simulink model "Horizontal1804"  (R2026b)
settings: Solver=FixedStepDiscrete  StopTime=inf  FixedStep=Official.Step
PostLoadFcn:
  | run(fullfile(fileparts(get_param('StampFly_IMU400','FileName')),'config','startup.m'));
InitFcn:
  | init_imu_flight;
undefined symbols (not defined in the file): Official
libraries: slpidlib x7, simulink x4, mspfiltlib x1
(part 1 of 5)
settings Model: SILPILModeSetting=veronly  Creator=tyasukaw  LastModifiedBy=tyasukaw
settings SolverCC: AutoInsertRateTranBlk=on
settings OptimizationCC: DifferentSizesBufferReuse=on  EfficientTunableParamExpr=on  EnhancedBackFolding=on  MaxStackSize=64  OptimizationCustomize=off  OptimizeBlockOrder=speed  PassReuseOutputArgsAs=Individual arguments  RemoveInternalMemoryZeroInit=on  RemoveRootLevelIOMemoryZeroInit=on
settings DebuggingCC: ParameterTunabilityLossMsg=error
settings HardwareCC: ProdHWDeviceType=ARM Compatible->ARM Cortex  ProdLargestAtomicFloat=Double  ProdLargestAtomicInteger=Long
settings SFSimCC: MATLABDynamicMemAlloc=off
settings RTWCC: BuildConfiguration=Faster Runs  DataTypeReplacement=CDataTypesFixedWidth  Description=Embedded Coder  HardwareBoard=ESP32-S3 Series (Arduino Compatible)  SystemTargetFile=ert.tlc  TLCOptions="-aInlineSetEventsForThisBaseRateFcn=TLC_FALSE -aSuppressMultiTaskScheduler=TLC_FALSE  -aRateBasedStepFcn=0"  TemplateMakefile=ert_default_tmf  Toolchain=ESP32
settings CodeAppCC: ForceParamTrailComments=on  IgnoreCustomStorageClasses=off  InsertBlockDesc=on  OperatorAnnotations=on  SFDataObjDesc=on  SimulinkDataObjDesc=on
settings ERTTargetCC: CombineSignalStateStructs=on  ExtModeAutomaticAllocSize=off  ExtModeIntrfLevel=Level2 - Open  ExtModeMexFile=ext_xcp  ExtModeStaticAlloc=on  MaxIdInt16=INT16_MAX  MaxIdInt32=INT32_MAX  MaxIdInt64=INT64_MAX  MaxIdInt8=INT8_MAX  MaxIdUint16=UINT16_MAX  MaxIdUint32=UINT32_MAX  MaxIdUint64=UINT64_MAX  MaxIdUint8=UINT8_MAX  MinIdInt16=INT16_MIN  MinIdInt32=INT32_MIN  MinIdInt64=INT64_MIN  MinIdInt8=INT8_MIN  SupportContinuousTime=on  SupportVariableSizeSignals=on

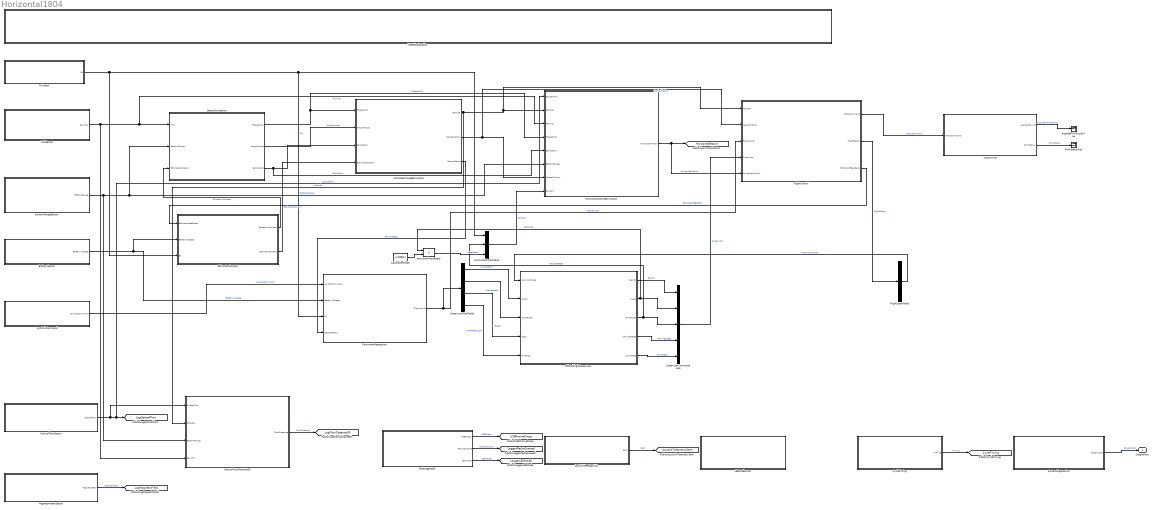
== system Horizontal1804 ==
  AppliedPWMCountsTap : Terminator
      settings: Description=AppliedPWMCountsTap：使用しない観測出力をここで終端します。接続された制御信号を変更しません。
  AttitudeAltitudeEstimation : Subsystem  Description=IMU Filter で姿勢・補正済み角速度、MATLAB Function の AltitudeKalman で高度・鉛直速度を推定します。状態フラグと推定診断をまとめ、ログ用 Goto をこの階層から公開します。
      mask help: IMU Filter で姿勢・補正済み角速度、MATLAB Function の AltitudeKalman で高度・鉛直速度を推定します。状態フラグと推定診断をまとめ、ログ用 Goto をこの階層から公開します。
      mask Display: disp('AttitudeAltitudeEstimation');port_label('input',1,'FilteredIMU');port_label('input',2,'HeightInputs');port_label('input',3,'Calibration');port_label('input',4,'EstimatorContext');port_label('output',1,'Attitude');port_label('output',2,'VerticalMotion');port_label('output',3,'SensorStatus');
  BatterySensor : Subsystem  Description=電池電圧 [V] と読み出し有効性を取得します。I2C 使用中は前回値を保持し、ReadValid=0 を公開します。
      mask help: 電池電圧 [V] と読み出し有効性を取得します。I2C 使用中は前回値を保持し、ReadValid=0 を公開します。
      mask Display: disp('BatterySensor');port_label('output',1,'BatteryVoltage');
  BottomRangeSensor : Subsystem  Description=下向き ToF の初期化完了後は Mode に依存せず取得します。距離 [mm] と Fresh を BottomRange バスへまとめ、Status と診断は Goto で公開します。Fresh は 400 Hz の読み出しではなく新しい測定結果の到着を示します。前方センサーは未使用です。
      mask help: 下向き ToF の初期化完了後は Mode に依存せず取得します。距離 [mm] と Fresh を BottomRange バスへまとめ、Status と診断は Goto で公開します。Fresh は 400 Hz の読み出しではなく新しい測定結果の到着を示します。前方センサーは未使用です。
      mask Display: disp('BottomRangeSensor');port_label('output',1,'BottomRange');
  CalibrationMode : Constant  Description=CalibrationMode：水平推定・制御のデータと実行条件を選択・結合します。2軸の順序は局所X（基準機首）、Y（右）です。  Value=uint8(1)
  CommandPreparation : Subsystem  Description=操縦指令、電池電圧、実測 dt、センサーフラグを名前付きバスへまとめます。Stateflow と飛行制御へ同じ入力を渡し、ログ用の観測も公開します。
      mask help: 操縦指令、電池電圧、実測 dt、センサーフラグを名前付きバスへまとめます。Stateflow と飛行制御へ同じ入力を渡し、ログ用の観測も公開します。
      mask Display: disp('CommandPreparation');port_label('input',1,'JoystickCommand');port_label('input',2,'BatteryVoltage');port_label('input',3,'Dt');port_label('input',4,'SensorStatus');port_label('output',1,'FlightInputs');
  CycleTiming : Subsystem  Description=ログとモーター適用後の処理時間・周期間隔を観測します。制御値を変更せず、計測位置を信号依存で固定します。
      mask help: ログとモーター適用後の処理時間・周期間隔を観測します。制御値を変更せず、計測位置を信号依存で固定します。
      mask Display: disp('CycleTiming');port_label('output',1,'Timing');
  DataLogging50 : Subsystem  Description=全ログ入力を50 Hzで同時に保存し、400 Hzタスク内で指令補足を2.5 ms後、センサー補足を5 ms後、通常ログを10 ms後に作成・送信します。水平補足は7.5 ms後です。保存時刻・Sequence・項目順・型・CRCで対応づけます。Channelは操縦受信・ログ受信機と同じ専用CHです。
      mask help: 生センサー・推定・制御・追加センサーを名前付き From で取得し、50 Hz の SFI8/SFIX/SFIY ログを生成して送信します。型・順序・CRC は維持します。Channel は RadioUSBTransport50 の設定画面で操縦側と揃えます。
      mask Display: disp('DataLogging50');port_label('output',1,'USBDrops');port_label('output',2,'RadioQueued');port_label('output',3,'LEDMode');
  EstimatorContext : Subsystem  Description=前周期のモード、高度制御許可、姿勢・待機リセットを 1 周期保持して推定器へ渡します。状態更新順序と代数ループ回避に必要な遅延です。
      mask help: 前周期のモード、高度制御許可、姿勢・待機リセットを 1 周期保持して推定器へ渡します。状態更新順序と代数ループ回避に必要な遅延です。
      mask Display: disp('EstimatorContext');port_label('input',1,'EstimatorFeedback');port_label('input',2,'BatteryVoltage');port_label('input',3,'Dt');port_label('output',1,'CorrectionContext');port_label('output',2,'EstimatorContext');
  FlightControl : Subsystem  Description=最上位 Stateflow の指令と姿勢・高度を受け、離着陸、7 個の PID、モーター配分を計算します。出力は Duty・PWM Counts、飛行状態、次周期の推定器コンテキストです。状態ログもこの階層に含みます。
      mask help: 最上位 Stateflow の指令と姿勢・高度を受け、離着陸、7 個の PID、モーター配分を計算します。出力は Duty・PWM Counts、飛行状態、次周期の推定器コンテキストです。状態ログもこの階層に含みます。
      mask Display: disp('FlightControl');port_label('input',1,'Attitude');port_label('input',2,'VerticalMotion');port_label('input',3,'FlightInputs');port_label('input',4,'Supervisor');port_label('input',5,'HorizontalMotion');port_label('output',1,'MotorCommand');port_label('output',2,'FlightStatus');port_label('output',3,'EstimatorFeedback');
  FlightStateFields : BusSelector  Description=FlightStateFields：バスから PreviousMode を選びます。元のベクトルの成分順序は変更しません。  OutputSignals=PreviousMode
  HorizontalContextBus : BusCreator  Description=HorizontalContextBus：水平推定・制御のデータと実行条件を選択・結合します。2軸の順序は局所X（基準機首）、Y（右）です。  Inputs=3  OutDataTypeStr=Bus: HorizontalContextBus  NonVirtualBus=on
      settings: InheritFromInputs=off
  HorizontalMotionEstimation : Subsystem  Description=HorizontalMotionEstimation：水平推定・制御のデータと実行条件を選択・結合します。2軸の順序は局所X（基準機首）、Y（右）です。
      mask help: 水平推定：フロー時刻に同期した角速度積分、ToFと姿勢による投影、品質と鮮度の確認を行います。局所Xは基準機首、Yは右です。
      mask Display: disp('HorizontalMotionEstimation');port_label('input',1,'OpticalFlow');port_label('input',2,'Attitude');port_label('input',3,'RawIMU');port_label('input',4,'FilteredIMU');port_label('input',5,'Calibration');port_label('input',6,'BottomRange');port_label('input',7,'VerticalMotion');port_label('input',8,'Context');port_label('output',1,'HorizontalMotion');
  HorizontalPoseReady : RelationalOperator  Description=HorizontalPoseReady：水平推定・制御のデータと実行条件を選択・結合します。2軸の順序は局所X（基準機首）、Y（右）です。  Operator=>  OutDataTypeStr=boolean  RndMeth=Simplest  InputSameDT=off
  IMUSensor : Subsystem  Description=BMI270 の生加速度・角速度を XYZ のままバスへまとめます。センサー座標であり、単位は m/s²・rad/s。温度と Fresh は名前付き Goto でログへ公開します。
      mask help: BMI270 の生加速度・角速度を XYZ のままバスへまとめます。センサー座標であり、単位は m/s²・rad/s。温度と Fresh は名前付き Goto でログへ公開します。
      mask Display: disp('IMUSensor');port_label('output',1,'RawIMU');
  JoystickCommand : Subsystem  Description=公式 JoyStick から通常飛行の指令を受信し、操縦バスと診断を公開します。Flip 用押し込みボタンは使用しません。専用 Channel は内部の BasicJoystick で設定します。
      mask help: 公式 JoyStick から通常飛行の指令を受信し、操縦バスと診断を公開します。Flip 用押し込みボタンは使用しません。専用 Channel は内部の BasicJoystick で設定します。
      mask Display: disp('JoystickCommand');port_label('output',1,'JoystickCommand');
  JoystickFeedback40 : Subsystem  Description=公式 JoyStick の画面へ姿勢・高度・電池・制御状態を 40 Hz で返信します。通常ログとは別の公式 120 byte 形式です。
      mask help: 公式 JoyStick の画面へ姿勢・高度・電池・制御状態を 40 Hz で返信します。通常ログとは別の公式 120 byte 形式です。
      mask Display: disp('JoystickFeedback40');port_label('output',1,'Sent');
  LEDAndBuzzer : Subsystem  Description=飛行状態・電池・通信・姿勢リセット要求から LED と音を決め、出力キューへ渡します。機体ボタンの押下・解放による再起動もここで扱います。
      mask help: 飛行状態・電池・通信・姿勢リセット要求から LED と音を決め、出力キューへ渡します。機体ボタンの押下・解放による再起動もここで扱います。
      mask Display: disp('LEDAndBuzzer');
  MagnetometerSensor : Subsystem  Description=BMM150 の磁場 XYZ [μT] と有効性・Fresh・診断を取得します。センサー座標を保ってログへ渡し、姿勢推定・制御には使いません。
      mask help: BMM150 の磁場 XYZ [μT] と有効性・Fresh・診断を取得します。センサー座標を保ってログへ渡し、姿勢推定・制御には使いません。
      mask Display: disp('MagnetometerSensor');port_label('output',1,'MagneticField');
  ModelExplanation : Subsystem  Description=StampFly の学習用実装。400 Hz でセンサー取得→校正→姿勢・高度推定→離着陸と 7 PID→4 モーターへ処理します。Flip はありません。最上位 Stateflow がモードを管理し、下段は観測・記録・状態表示です。
      mask help: StampFly の学習用実装。400 Hz でセンサー取得→校正→姿勢・高度推定→離着陸と 7 PID→4 モーターへ処理します。Flip はありません。最上位 Stateflow がモードを管理し、下段は観測・記録・状態表示です。
      mask Display: disp(sprintf('StampFly IMU Filter / 400 Hz\nセンサー取得 → 校正・前処理 → 姿勢・高度推定 → PID → モーター\n飛行モードは最上位のStateflowで管理。下段は観測・記録・状態表示。'));
  MotorWrite : Subsystem  Description=8 bit の Counts を実機モーターへ適用します。順序 [FR, FL, RR, RL]、GPIO [42, 5, 41, 10]、150 kHz 指定です。実適用 Counts と PWM 診断を Goto で公開します。
      mask help: 8 bit の Counts を実機モーターへ適用します。順序 [FR, FL, RR, RL]、GPIO [42, 5, 41, 10]、150 kHz 指定です。実適用 Counts と PWM 診断を Goto で公開します。
      mask Display: disp('MotorWrite');port_label('input',1,'MotorCommand');port_label('output',1,'AppliedCounts');port_label('output',2,'PWMStatus');
  OfficialFlightSupervisor : Stateflow chart  Description=最上位の飛行状態管理です。前周期 Mode、操縦ボタン、新パケット、異常フラグ、姿勢リセットを受け、校正・待機・飛行・着陸の分岐と推定器リセットを決めます。  TreatAsAtomicUnit=on
      mask help: 最上位の飛行状態管理です。前周期 Mode、操縦ボタン、新パケット、異常フラグ、姿勢リセットを受け、校正・待機・飛行・着陸の分岐と推定器リセットを決めます。
  OpticalFlowDistance50 : Subsystem  Description=生の累積光学フロー、姿勢、角速度、下向き ToF から平面上の東・北移動距離を 50 Hz で作ります。回転補償と品質判定を行い、無効な区間は位置を保持します。385 count/rad は初期値です。
      mask help: 生の累積光学フロー、姿勢、角速度、下向き ToF から平面上の東・北移動距離を 50 Hz で作ります。回転補償と品質判定を行い、無効な区間は位置を保持します。385 count/rad は初期値です。
      mask Display: disp('OpticalFlowDistance50');port_label('input',1,'OpticalFlow');port_label('input',2,'Attitude');port_label('input',3,'BottomRange');port_label('input',4,'RawIMU');port_label('output',1,'FlowDistance');
  OpticalFlowSensor : Subsystem  Description=PMW3901 の生 2 軸差分・品質・診断・累積カウントを取得します。表示・記録専用で、水平位置制御へは戻しません。
      mask help: PMW3901 の生 2 軸差分・品質・診断・累積カウントを取得します。表示・記録専用で、水平位置制御へは戻しません。
      mask Display: disp('OpticalFlowSensor');port_label('output',1,'OpticalFlow');
  PWMStatusTap : Terminator
      settings: Description=PWMStatusTap：使用しない観測出力をここで終端します。接続された制御信号を変更しません。
  SensorCorrection : Subsystem  Description=センサー座標から機体 XYZ へ変換し、800 周期の静止校正とフィルターを行います。加速度 XYZ・角速度 XYZ の順を維持し、ToF の保持・外れ値処理と鉛直加速度もまとめます。推定用の前処理は Mode 0, 1 で保持します。
      mask help: センサー座標から機体 XYZ へ変換し、800 周期の静止校正とフィルターを行います。加速度 XYZ・角速度 XYZ の順を維持し、ToF の保持・外れ値処理と鉛直加速度もまとめます。推定用の前処理は Mode 0, 1 で保持します。
      mask Display: disp('SensorCorrection');port_label('input',1,'IMU');port_label('input',2,'BottomRange');port_label('input',3,'EstimatorContext');port_label('output',1,'FilteredIMU');port_label('output',2,'HeightInputs');port_label('output',3,'Calibration');
  SupervisorCommandBus : BusCreator  Description=SupervisorCommandBus：異なる単位・型を持つ関連信号を名前付きバスにまとめます。入力線の信号名が項目名です。  Inputs=5
  SupervisorPilotFields : BusSelector  Description=SupervisorPilotFields：バスから ArmButton,NewPacket,Flags,AHRSRequest を選びます。元のベクトルの成分順序は変更しません。  OutputSignals=ArmButton,NewPacket,Flags,AHRSRequest
  SystemDiagnostics : Subsystem  Description=各機能の診断 From を型付き名前付きバスへまとめます。50 Hz/40 Hz の値を必要な箇所で保持し、全体の診断出力へ渡します。
      mask help: 各機能の診断 From を型付き名前付きバスへまとめます。50 Hz/40 Hz の値を必要な箇所で保持し、全体の診断出力へ渡します。
      mask Display: disp('SystemDiagnostics');port_label('output',1,'Diagnostics');
  TickStart : Subsystem  Description=400 Hz 周期の開始時刻、実測 dt、タイマー診断を取得し、秒への時刻変換と Goto 公開をこの階層でまとめます。
      mask help: 400 Hz 周期の開始時刻、実測 dt、タイマー診断を取得し、秒への時刻変換と Goto 公開をこの階層でまとめます。
      mask Display: disp('TickStart');port_label('output',1,'Dt');
  Diagnostics : Outport  OutDataTypeStr=Bus: OfficialDiagnosticBus  BusOutputAsStruct=on
  tag scope: CycleTiming=global, HorizontalMotion=global, JoystickTelemetrySent=global, LogFlowDistance50=global, LogMagneticField=global, LogOpticalFlow=global, LoggerLEDMode=global, LoggerRadioQueued=global, USBFrameDrops=global
  wires:
  JoystickFeedback40/1(Sent) -> [JoystickTelemetrySent]  "Sent"
  CycleTiming/1(Timing) -> [CycleTiming]  "Timing"
  SystemDiagnostics/1(Diagnostics) -> Diagnostics/1  "Diagnostics"
  DataLogging50/1(USBDrops) -> [USBFrameDrops]  "USBDrops"
  DataLogging50/2(RadioQueued) -> [LoggerRadioQueued]  "RadioQueued"
  DataLogging50/3(LEDMode) -> [LoggerLEDMode]  "LEDMode"
  SupervisorCommandBus/1 -> FlightControl/4(Supervisor)  "Supervisor"
  OfficialFlightSupervisor/5(connected) -> SupervisorCommandBus/5  "Connected"
  OfficialFlightSupervisor/4(parkingReset) -> SupervisorCommandBus/4  "ParkingReset"
  OfficialFlightSupervisor/1(branch) -> SupervisorCommandBus/1  "Branch"
  SupervisorPilotFields/4 -> OfficialFlightSupervisor/5(ahrsFlag)  "<AHRSRequest>"
  SupervisorPilotFields/3 -> OfficialFlightSupervisor/4(flags)  "<Flags>"
  SupervisorPilotFields/2 -> OfficialFlightSupervisor/3(newPacket)  "<NewPacket>"
  SupervisorPilotFields/1 -> OfficialFlightSupervisor/2(button)  "<ArmButton>"
  FlightStateFields/1 -> OfficialFlightSupervisor/1(previousMode)  "<PreviousMode>"
  FlightControl/2(FlightStatus) -> FlightStateFields/1  "FlightStatus"
  FlightControl/1(MotorCommand) -> MotorWrite/1(MotorCommand)  "MotorCommand"
  MotorWrite/1(AppliedCounts) -> AppliedPWMCountsTap/1  "AppliedPWMCounts"
  MotorWrite/2(PWMStatus) -> PWMStatusTap/1  "PWMStatus"
  AttitudeAltitudeEstimation/3(SensorStatus) -> CommandPreparation/4(SensorStatus)  "SensorStatus"
  CommandPreparation/1(FlightInputs) -> SupervisorPilotFields/1, FlightControl/3(FlightInputs)  "FlightInputs"
  JoystickCommand/1(JoystickCommand) -> CommandPreparation/1(JoystickCommand)  "JoystickCommand"
  FlightControl/3(EstimatorFeedback) -> EstimatorContext/1(EstimatorFeedback)  "EstimatorFeedback"
  EstimatorContext/2(EstimatorContext) -> AttitudeAltitudeEstimation/4(EstimatorContext)  "EstimatorContext"
  OpticalFlowDistance50/1(FlowDistance) -> [LogFlowDistance50]  "FlowDistance"
  MagnetometerSensor/1(MagneticField) -> [LogMagneticField]  "MagneticField"
  CalibrationMode/1 -> HorizontalPoseReady/2
  EstimatorContext/1(CorrectionContext) -> SensorCorrection/3(EstimatorContext)  "CorrectionContext"
  BatterySensor/1(BatteryVoltage) -> CommandPreparation/2(BatteryVoltage), EstimatorContext/2(BatteryVoltage)  "BatteryVoltage"
  OfficialFlightSupervisor/2(mode) -> SupervisorCommandBus/2, HorizontalPoseReady/1  "PreMode"
  SensorCorrection/2(HeightInputs) -> AttitudeAltitudeEstimation/2(HeightInputs)  "HeightInputs"
  HorizontalMotionEstimation/1(HorizontalMotion) -> [HorizontalMotion], FlightControl/5(HorizontalMotion)  "HorizontalMotion"
  AttitudeAltitudeEstimation/2(VerticalMotion) -> FlightControl/2(VerticalMotion), HorizontalMotionEstimation/7(VerticalMotion)  "VerticalMotion"
  SensorCorrection/1(FilteredIMU) -> AttitudeAltitudeEstimation/1(FilteredIMU), HorizontalMotionEstimation/4(FilteredIMU)  "FilteredIMU"
  SensorCorrection/3(Calibration) -> AttitudeAltitudeEstimation/3(Calibration), HorizontalMotionEstimation/5(Calibration)  "Calibration"
  BottomRangeSensor/1(BottomRange) -> HorizontalMotionEstimation/6(BottomRange), SensorCorrection/2(BottomRange), OpticalFlowDistance50/3(BottomRange)  "BottomRange"
  OpticalFlowSensor/1(OpticalFlow) -> HorizontalMotionEstimation/1(OpticalFlow), [LogOpticalFlow], OpticalFlowDistance50/1(OpticalFlow)  "OpticalFlow"
  IMUSensor/1(RawIMU) -> SensorCorrection/1(IMU), HorizontalMotionEstimation/3(RawIMU), OpticalFlowDistance50/4(RawIMU)  "RawIMU"
  AttitudeAltitudeEstimation/1(Attitude) -> FlightControl/1(Attitude), HorizontalMotionEstimation/2(Attitude), OpticalFlowDistance50/2(Attitude)  "Attitude"
  HorizontalContextBus/1 -> HorizontalMotionEstimation/8(Context)  "Context"
  TickStart/1(Dt) -> CommandPreparation/3(Dt), HorizontalContextBus/1, EstimatorContext/3(Dt)  "Dt"
  OfficialFlightSupervisor/3(ahrsReset) -> SupervisorCommandBus/3, HorizontalContextBus/2  "AttitudeReset"
  HorizontalPoseReady/1 -> HorizontalContextBus/3  "PoseReady"

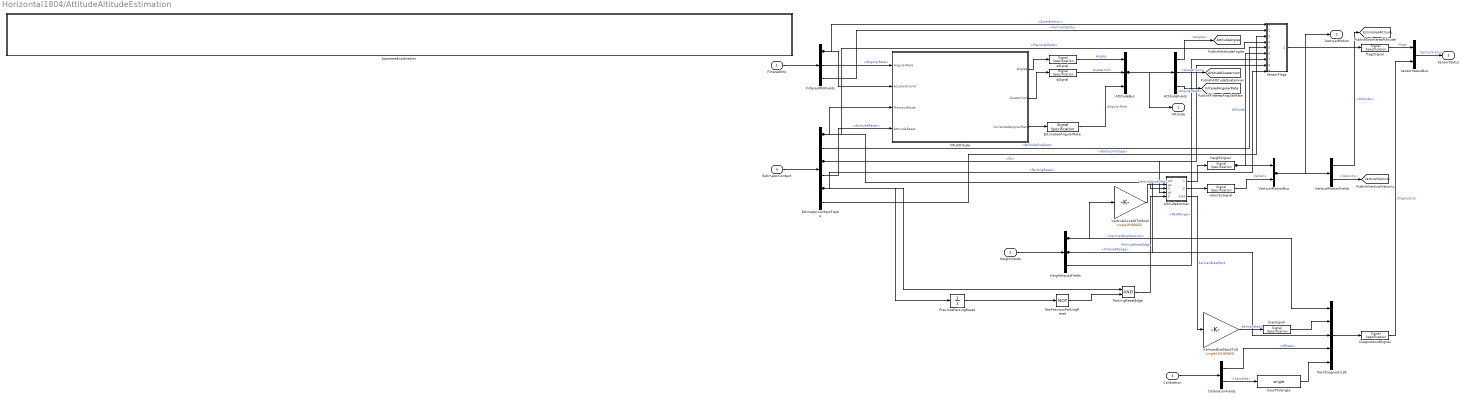
== system Horizontal1804/AttitudeAltitudeEstimation ==
  FilteredIMU : Inport
  HeightInputs : Inport  Port=2
  Calibration : Inport  Port=3
  EstimatorContext : Inport  Port=4
  AltitudeKalman : MATLAB Function  Description=ToF高さ[m]と鉛直加速度[m/s²]から[速度m/s;高度m;加速度バイアスm/s²]を推定するMATLAB Functionです。加速度のg換算と待機リセットの立上りは周囲のブロックで明示します。高度・速度は既存PIDへ直接渡します。  TreatAsAtomicUnit=on
  AttitudeBus : BusCreator  Description=AttitudeBus：異なる単位・型を持つ関連信号を名前付きバスにまとめます。入力線の信号名が項目名です。  Inputs=3
  AttitudeFields : BusSelector  Description=AttitudeFields：バスから Angles,Quaternion,AngularRate を選びます。元のベクトルの成分順序は変更しません。  OutputSignals=Angles,Quaternion,AngularRate
  CalibrationFields : BusSelector  Description=CalibrationFields：バスから Offsets,Samples を選びます。元のベクトルの成分順序は変更しません。  OutputSignals=Offsets,Samples
  CountToSingle : DataTypeConversion  Description=CountToSingle：後段のバス・演算に合わせて single 型へ変換します。  OutDataTypeStr=single  SaturateOnIntegerOverflow=off  RndMeth=Floor
  Diagnostics8Signal : SignalSpecification  OutDataTypeStr=single  Dimensions=8
  EstimatedAngularRate : SignalSpecification  OutDataTypeStr=single  Dimensions=3
  EstimatorContextFields : BusSelector  Description=EstimatorContextFields：バスから PreviousMode,AltitudeEnabled,Dt,AttitudeReset,ParkingReset,BatteryVoltage を選びます。元のベクトルの成分順序は変更しません。  OutputSignals=PreviousMode,AltitudeEnabled,Dt,AttitudeReset,ParkingReset,BatteryVoltage
  FilteredIMUFields : BusSelector  Description=FilteredIMUFields：バスから Acceleration,AngularRate,VerticalDelta を選びます。元のベクトルの成分順序は変更しません。  OutputSignals=Acceleration,AngularRate,VerticalDelta
  HeightInputsFields : BusSelector  Description=HeightInputsFields：バスから VerticalAcceleration,FilteredRange,RawRange を選びます。元のベクトルの成分順序は変更しません。  OutputSignals=VerticalAcceleration,FilteredRange,RawRange
  IMUAttitude : Subsystem  Description=機体 XYZ と推定器座標の変換、標準 IMU Filter、制御用の姿勢と角速度への変換をまとめます。停止中の保持と再開時リセットを行います。
      mask help: 機体 XYZ と推定器座標の変換、標準 IMU Filter、制御用の姿勢と角速度への変換をまとめます。停止中の保持と再開時リセットを行います。
      mask Display: disp('IMUAttitude');port_label('input',1,'AngularRate');port_label('input',2,'AccelerationG');port_label('input',3,'PreviousMode');port_label('input',4,'AttitudeReset');port_label('output',1,'Angles');port_label('output',2,'Quaternion');port_label('output',3,'CorrectedAngularRate');
  JapaneseExplanation : Subsystem  Description=IMU Filter で姿勢・補正済み角速度、MATLAB Function の AltitudeKalman で高度・鉛直速度を推定します。状態フラグと推定診断をまとめ、ログ用 Goto をこの階層から公開します。
      mask help: IMU Filter で姿勢・補正済み角速度、MATLAB Function の AltitudeKalman で高度・鉛直速度を推定します。状態フラグと推定診断をまとめ、ログ用 Goto をこの階層から公開します。
      mask Display: disp(sprintf('IMU Filter で姿勢・補正済み角速度、MATLAB Function の AltitudeKalman で高度・鉛直速度を推\n定します。\n状態フラグと推定診断をまとめ、ログ用 Goto をこの階層から公開します。'));
  KalmanBiasMps2ToG : Gain  Description=推定器内の加速度バイアス[m/s²]を従来ログのgへ換算します。制御用の高度・速度には影響しません。  Gain=single(1/9.80665)  OutDataTypeStr=single
  NotPreviousParkingReset : Logic  Description=前周期に待機リセットが要求されていなかったことを確認します。  Operator=NOT  IconShape=distinctive  AllPortsSameDT=off  OutDataTypeStr=boolean
  PackDiagnostics8 : Mux  Description=PackDiagnostics8：同じ型の値を入力端子の順でベクトルに結合します。ログ仕様・モーター順に対応する結合は順序を保ちます。  Inputs=5
  ParkingResetEdge : Logic  Description=待機へ入る立上りだけでカルマン共分散を初期化します。待機中の毎周期リセットによる飛行切替直後の速度ジャンプを防ぎます。  IconShape=distinctive  AllPortsSameDT=off  OutDataTypeStr=boolean
  PreviousParkingReset : UnitDelay  Description=前周期の待機リセット要求を記憶し、待機へ入る瞬間だけを検出します。  InitialCondition=false  SampleTime=.0025
  SensorFlags : MATLAB Function  Description=推定・状態管理で使う [過大加速度; 距離異常の継続回数; 低電圧の継続回数] を uint8 で出力します。短い揺れを平滑化し、距離は最大 20 回、低電圧は最大 100 回まで数えます。  TreatAsAtomicUnit=on
  SensorStatusBus : BusCreator  Description=SensorStatusBus：異なる単位・型を持つ関連信号を名前付きバスにまとめます。入力線の信号名が項目名です。  Inputs=2
  VerticalAccelGToMps2 : Gain  Description=鉛直加速度をgからm/s²へ換算します。高度[m]・速度[m/s]の予測に使うため、推定器入口で単位をそろえます。  Gain=single(9.80665)  OutDataTypeStr=single
  VerticalMotionBus : BusCreator  Description=VerticalMotionBus：異なる単位・型を持つ関連信号を名前付きバスにまとめます。入力線の信号名が項目名です。  Inputs=2
  VerticalMotionFields : BusSelector  Description=VerticalMotionFields：バスから Altitude,Velocity を選びます。元のベクトルの成分順序は変更しません。  OutputSignals=Altitude,Velocity
  aSignal : SignalSpecification  OutDataTypeStr=single  Dimensions=3
  biasSignal : SignalSpecification  OutDataTypeStr=single  Dimensions=1
  flagsSignal : SignalSpecification  OutDataTypeStr=uint8  Dimensions=3
  heightSignal : SignalSpecification  OutDataTypeStr=single  Dimensions=1
  qSignal : SignalSpecification  OutDataTypeStr=single  Dimensions=4
  velocitySignal : SignalSpecification  OutDataTypeStr=single  Dimensions=1
  Attitude : Outport
  VerticalMotion : Outport  Port=2
  SensorStatus : Outport  Port=3
  tag scope: AttitudeAngles=global, AttitudeQuaternion=global, EstimatedAltitude=global, FilteredAngularRate=global, VerticalVelocity=global
  wires:
  HeightInputs/1 -> HeightInputsFields/1
  EstimatorContext/1 -> EstimatorContextFields/1
  Calibration/1 -> CalibrationFields/1
  FilteredIMU/1 -> FilteredIMUFields/1
  FilteredIMUFields/3 -> SensorFlags/2(arg_azd)  "<VerticalDelta>"
  EstimatorContextFields/3 -> SensorFlags/8(arg_dt), AltitudeKalman/4(dt)  "<Dt>"
  EstimatedAngularRate/1 -> AttitudeBus/3  "AngularRate"
  EstimatorContextFields/6 -> SensorFlags/3(arg_voltage)  "<BatteryVoltage>"
  FilteredIMUFields/2 -> IMUAttitude/1(AngularRate)  "<AngularRate>"
  EstimatorContextFields/2 -> SensorFlags/5(arg_altFlag)  "<AltitudeEnabled>"
  EstimatorContextFields/5 -> PreviousParkingReset/1, ParkingResetEdge/1, SensorFlags/9(arg_parkingReset)  "<ParkingReset>"
  FilteredIMUFields/1 -> SensorFlags/1(arg_accel), IMUAttitude/2(AccelerationG)  "<Acceleration>"
  EstimatorContextFields/1 -> SensorFlags/4(arg_mode), AltitudeKalman/3(mode), IMUAttitude/3(PreviousMode)  "<PreviousMode>"
  EstimatorContextFields/4 -> IMUAttitude/4(AttitudeReset)  "<AttitudeReset>"
  HeightInputsFields/1 -> PackDiagnostics8/1, VerticalAccelGToMps2/1  "<VerticalAcceleration>"
  IMUAttitude/1(Angles) -> aSignal/1
  HeightInputsFields/2 -> AltitudeKalman/1(alt), PackDiagnostics8/3  "<FilteredRange>"
  IMUAttitude/2(Quaternion) -> qSignal/1
  HeightInputsFields/3 -> SensorFlags/7(arg_rawRange)  "<RawRange>"
  IMUAttitude/3(CorrectedAngularRate) -> EstimatedAngularRate/1
  PackDiagnostics8/1 -> Diagnostics8Signal/1
  PreviousParkingReset/1 -> NotPreviousParkingReset/1
  aSignal/1 -> AttitudeBus/1  "Angles"
  SensorStatusBus/1 -> SensorStatus/1  "SensorStatus"
  VerticalMotionFields/1 -> [EstimatedAltitude]  "<Altitude>"
  qSignal/1 -> AttitudeBus/2  "Quaternion"
  NotPreviousParkingReset/1 -> ParkingResetEdge/2
  CalibrationFields/2 -> CountToSingle/1  "<Samples>"
  AttitudeFields/3 -> [FilteredAngularRate]  "<AngularRate>"
  AttitudeBus/1 -> Attitude/1, AttitudeFields/1
  VerticalMotionFields/2 -> [VerticalVelocity]  "<Velocity>"
  VerticalAccelGToMps2/1 -> AltitudeKalman/2(az)  "VerticalAccelMps2"
  ParkingResetEdge/1 -> AltitudeKalman/5(parkingReset)  "ParkingResetEdge"
  Diagnostics8Signal/1 -> SensorStatusBus/2  "Diagnostics"
  AttitudeFields/1 -> [AttitudeAngles]  "<Angles>"
  CountToSingle/1 -> PackDiagnostics8/5
  CalibrationFields/1 -> PackDiagnostics8/4  "<Offsets>"
  AttitudeFields/2 -> [AttitudeQuaternion]  "<Quaternion>"
  AltitudeKalman/1(height) -> heightSignal/1
  AltitudeKalman/2(velocity) -> velocitySignal/1
  AltitudeKalman/3(bias) -> KalmanBiasMps2ToG/1  "KalmanBiasMps2"
  heightSignal/1 -> VerticalMotionBus/1, SensorFlags/6(arg_height)  "Altitude"
  velocitySignal/1 -> VerticalMotionBus/2  "Velocity"
  KalmanBiasMps2ToG/1 -> biasSignal/1  "KalmanBiasG"
  SensorFlags/1(arg_flags) -> flagsSignal/1
  biasSignal/1 -> PackDiagnostics8/2
  VerticalMotionBus/1 -> VerticalMotion/1, VerticalMotionFields/1
  flagsSignal/1 -> SensorStatusBus/1  "Flags"

== system Horizontal1804/BatterySensor ==
  Battery : MATLABSystem  Description=機体の電池電圧 [V] と今回の読み出し成功 ReadValid を出力します。ToF・磁気と I2C の排他制御を共有し、使用中は待たずに前回値を返します。SampleTime は制御周期 0.0025 秒です。  Priority=4  System=official.Battery400  SampleTime=Official.Step  SimulateUsing=Code generation
      mask Type: official.Battery400
  BatteryVoltage : Outport
  tag scope: BatteryReadValid=global, BatteryVoltage=global
  wires:
  Battery/2 -> [BatteryReadValid]  "BatteryValid"
  Battery/1 -> BatteryVoltage/1, [BatteryVoltage]  "BatteryVoltage"

== system Horizontal1804/BottomRangeSensor ==
  BottomRangeBus : BusCreator  Description=BottomRangeBus：異なる単位・型を持つ関連信号を名前付きバスにまとめます。入力線の信号名が項目名です。  Inputs=2
  BottomToFSource : MATLABSystem  Description=初期化完了後は飛行モードに依存せず距離を取得します。距離 [mm]、Fresh、未使用の前方距離、Status、Info を出力します。I2C 読み出しは core0 の非同期処理で、400 Hz の制御は待ちません。推定側の校正・待機条件は別に管理します。  Priority=3  System=official.BottomToFSource  SampleTime=Official.Step  SimulateUsing=Code generation
      mask Type: official.BottomToFSource
  JapaneseExplanation : Subsystem  Description=下向き ToF の初期化完了後は Mode に依存せず取得します。距離 [mm] と Fresh を BottomRange バスへまとめ、Status と診断は Goto で公開します。Fresh は 400 Hz の読み出しではなく新しい測定結果の到着を示します。前方センサーは未使用です。
      mask help: 下向き ToF の初期化完了後は Mode に依存せず取得します。距離 [mm] と Fresh を BottomRange バスへまとめ、Status と診断は Goto で公開します。Fresh は 400 Hz の読み出しではなく新しい測定結果の到着を示します。前方センサーは未使用です。
      mask Display: disp(sprintf('下向き ToF の初期化完了後は Mode に依存せず取得します。\n距離 [mm] と Fresh を BottomRange バスへまとめ、Status と診断は Goto で公開します。\nFresh は 400 Hz の読み出しではなく新しい測定結果の到着を示します。\n前方センサーは未使用です。'));
  BottomRange : Outport
  tag scope: BottomDistanceMm=global, BottomRangeFresh=global, BottomRangeStatus=global, BottomToFDiagnostics=global, UnusedFrontRangeMm=global
  wires:
  BottomRangeBus/1 -> BottomRange/1  "BottomRange"
  BottomToFSource/5 -> [BottomToFDiagnostics]  "Info"
  BottomToFSource/4 -> [BottomRangeStatus]  "Status"
  BottomToFSource/3 -> [UnusedFrontRangeMm]  "FrontDistanceMm"
  BottomToFSource/2 -> BottomRangeBus/2, [BottomRangeFresh]  "Fresh"
  BottomToFSource/1 -> [BottomDistanceMm], BottomRangeBus/1  "DistanceMm"

== system Horizontal1804/CommandPreparation ==
  JoystickCommand : Inport
  BatteryVoltage : Inport  Port=2
  Dt : Inport  Port=3
  SensorStatus : Inport  Port=4
  CommandTapBus : BusCreator  Description=CommandTapBus：異なる単位・型を持つ関連信号を名前付きバスにまとめます。入力線の信号名が項目名です。  Inputs=2
  CommandTapFields : BusSelector  Description=CommandTapFields：バスから Sticks,AHRSRequest を選びます。元のベクトルの成分順序は変更しません。  OutputSignals=Sticks,AHRSRequest
  ControlInputs : BusCreator  Description=ControlInputs：異なる単位・型を持つ関連信号を名前付きバスにまとめます。入力線の信号名が項目名です。  Inputs=7
  JapaneseExplanation : Subsystem  Description=操縦指令、電池電圧、実測 dt、センサーフラグを名前付きバスへまとめます。Stateflow と飛行制御へ同じ入力を渡し、ログ用の観測も公開します。
      mask help: 操縦指令、電池電圧、実測 dt、センサーフラグを名前付きバスへまとめます。Stateflow と飛行制御へ同じ入力を渡し、ログ用の観測も公開します。
      mask Display: disp(sprintf('操縦指令、電池電圧、実測 dt、センサーフラグを名前付きバスへまとめます。\nStateflow と飛行制御へ同じ入力を渡し、ログ用の観測も公開します。'));
  JoystickCommandFields : BusSelector  Description=JoystickCommandFields：バスから Sticks,ArmButton,NewPacket,AHRSRequest を選びます。元のベクトルの成分順序は変更しません。  OutputSignals=Sticks,ArmButton,NewPacket,AHRSRequest
  SensorStatusFields : BusSelector  Description=SensorStatusFields：バスから Flags,Diagnostics を選びます。元のベクトルの成分順序は変更しません。  OutputSignals=Flags,Diagnostics
  SensorTapBus : BusCreator  Description=SensorTapBus：異なる単位・型を持つ関連信号を名前付きバスにまとめます。入力線の信号名が項目名です。  Inputs=2
  SensorTapFields : BusSelector  Description=SensorTapFields：バスから Flags,Diagnostics を選びます。元のベクトルの成分順序は変更しません。  OutputSignals=Flags,Diagnostics
  FlightInputs : Outport
  tag scope: AttitudeResetRequest=global, JoystickSticks=global, SensorDiagnostics=global, SensorFlags=global
  wires:
  ControlInputs/1 -> FlightInputs/1  "FlightInputs"
  CommandTapBus/1 -> CommandTapFields/1  "CommandTap"
  Dt/1 -> ControlInputs/6
  BatteryVoltage/1 -> ControlInputs/5
  CommandTapFields/2 -> [AttitudeResetRequest]  "<AHRSRequest>"
  SensorStatus/1 -> SensorStatusFields/1
  JoystickCommand/1 -> JoystickCommandFields/1
  JoystickCommandFields/4 -> CommandTapBus/2, ControlInputs/4  "<AHRSRequest>"
  JoystickCommandFields/3 -> ControlInputs/3  "<NewPacket>"
  JoystickCommandFields/2 -> ControlInputs/2  "<ArmButton>"
  JoystickCommandFields/1 -> CommandTapBus/1, ControlInputs/1  "<Sticks>"
  SensorTapFields/1 -> [SensorFlags]  "<Flags>"
  SensorStatusFields/1 -> ControlInputs/7, SensorTapBus/1  "<Flags>"
  SensorTapFields/2 -> [SensorDiagnostics]  "<Diagnostics>"
  SensorStatusFields/2 -> SensorTapBus/2  "<Diagnostics>"
  SensorTapBus/1 -> SensorTapFields/1  "SensorTap"
  CommandTapFields/1 -> [JoystickSticks]  "<Sticks>"

== system Horizontal1804/CycleTiming ==
  TimingEnd : MATLABSystem  Description=周期開始時刻からこの地点までの時間・周期間隔・平均・最大・超過などを記録します。IMU の Fresh、実適用 PWM、ログへの信号依存で計測位置を固定しています。全タスクの処理時間は生成 step のラッパーが別途計測します。  Priority=10000  System=official.TimingEnd400  SampleTime=Official.Step  SimulateUsing=Code generation
      mask Type: official.TimingEnd400
  Timing : Outport
  wires:
  [AppliedPWMCounts] -> TimingEnd/3
  [IMUSampleFresh] -> TimingEnd/2
  [CycleStartUs] -> TimingEnd/1
  TimingEnd/1 -> Timing/1  "Timing"
  [USBFrameDrops] -> TimingEnd/5
  [PWMStatus] -> TimingEnd/4

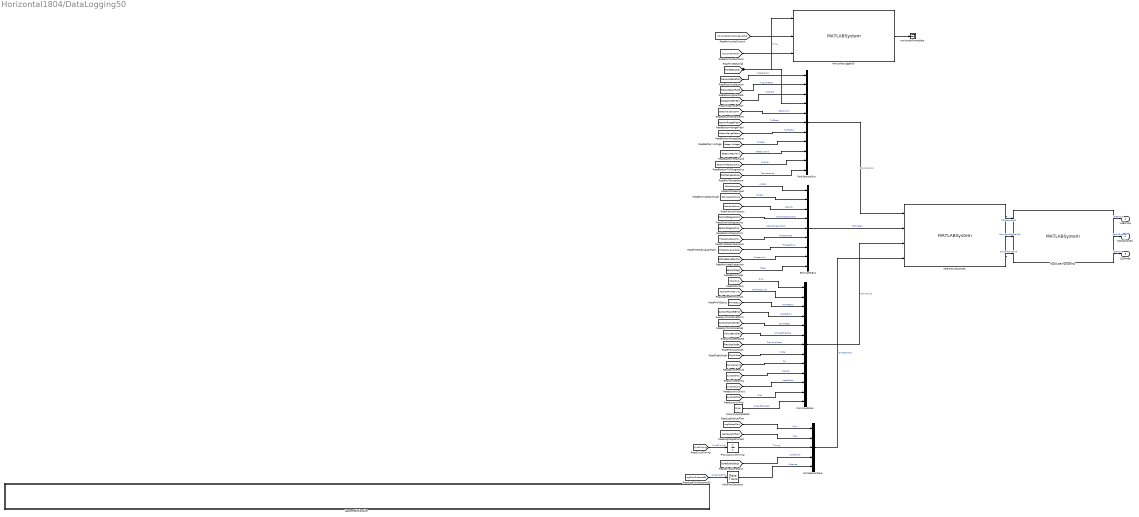
== system Horizontal1804/DataLogging50 ==
  CommandsBus : BusCreator  Description=CommandsBus：異なる単位・型を持つ関連信号を名前付きバスにまとめます。入力線の信号名が項目名です。  Inputs=13  OutDataTypeStr=Bus: BasicLogCommandBus  NonVirtualBus=on
  EstimatesBus : BusCreator  Description=EstimatesBus：異なる単位・型を持つ関連信号を名前付きバスにまとめます。入力線の信号名が項目名です。  Inputs=9  OutDataTypeStr=Bus: LogEstimateBus  NonVirtualBus=on
  ExtraSensorsBus : BusCreator  Description=ExtraSensorsBus：異なる単位・型を持つ関連信号を名前付きバスにまとめます。入力線の信号名が項目名です。  Inputs=5  OutDataTypeStr=Bus: LogExtraBus  NonVirtualBus=on
  HoldFlowDistance : RateTransition  OutPortSampleTime=.0025
  HorizontalFrameSent : Terminator
      settings: Description=HorizontalFrameSent：水平推定・制御のデータと実行条件を選択・結合します。2軸の順序は局所X（基準機首）、Y（右）です。
  HorizontalLogger50 : MATLABSystem  Description=50 Hzログと同じ時刻の水平診断を保存し、15 ms後にCRC作成、17.5 ms後に送信します。他のログ計算と重ならない400 Hz周期へ分散します。  System=horizontal.Logger  SimulateUsing=Code generation
      mask Type: horizontal.Logger
  JapaneseExplanation : Subsystem  Description=生センサー・推定・制御・追加センサーを名前付き From で取得し、50 Hz の SFI8/SFIX/SFIY ログを生成して送信します。型・順序・CRC は維持します。Channel は RadioUSBTransport50 の設定画面で操縦側と揃えます。
      mask help: 生センサー・推定・制御・追加センサーを名前付き From で取得し、50 Hz の SFI8/SFIX/SFIY ログを生成して送信します。型・順序・CRC は維持します。Channel は RadioUSBTransport50 の設定画面で操縦側と揃えます。
      mask Display: disp(sprintf('生センサー・推定・制御・追加センサーを名前付き From で取得し、50 Hz の SFI8/SFIX/SFIY ログ\nを生成して送信します。\n型・順序・CRC は維持します。\nChannel は RadioUSBTransport50 の設定画面で操縦側と揃えます。'));
  MotorOutputEnabled : Constant  Description=MotorOutputEnabled：固定値 true を出力します。意味と単位は親の機能説明と信号名を参照します。  Value=true  OutDataTypeStr=boolean
  PreviousCycleTiming : UnitDelay  Description=PreviousCycleTiming：前周期の値を保持して出力します。更新順序と状態保持に必要な 1 周期遅延です。初期値 zeros(8,1,'uint32')、周期 .0025 秒。  InitialCondition=zeros(8,1,'uint32')  SampleTime=.0025
  RadioUSBTransport50 : MATLABSystem  Description=完成した通常・指令・センサー補足を一度ずつ別周期でESP-NOW/USBキューへ送ります。Channelは操縦受信・ログ受信機と同じ専用CHです。  System=horizontal.TelemetryTransport  Channel=uint8(3)  SimulateUsing=Code generation
      mask Type: horizontal.TelemetryTransport
  RawSensorsBus : BusCreator  Description=RawSensorsBus：異なる単位・型を持つ関連信号を名前付きバスにまとめます。入力線の信号名が項目名です。  Inputs=11  OutDataTypeStr=Bus: LogRawBus  NonVirtualBus=on
  TelemetryPacker50 : MATLABSystem  Description=50 Hzで全ログ入力を同時に保存し、SFI8・SFIX・SFIYを別の400 Hz周期で作成します。保存時刻・Sequence・項目順・型・CRCは従来と同じです。  System=horizontal.TelemetryPacker  BuildID=uint32(1401)  FirmwareRevision=uint32(1804)  SimulateUsing=Code generation
      mask Type: horizontal.TelemetryPacker
  USBDrops : Outport
  RadioQueued : Outport  Port=2
  LEDMode : Outport  Port=3
  wires:
  [FlightMode] -> CommandsBus/8  "Mode"
  [BatteryReadValid] -> RawSensorsBus/9  "BatteryValid"
  [BottomRangeStatus] -> RawSensorsBus/7  "ToFStatus"
  [CycleTiming] -> PreviousCycleTiming/1  "CycleTiming"
  [LogOpticalFlow] -> ExtraSensorsBus/1  "Flow"
  [SensorDiagnostics] -> EstimatesBus/5  "SensorDiagnostics"
  [IMUSampleFresh] -> RawSensorsBus/3  "IMUFresh"
  [JoystickSticks] -> CommandsBus/11  "UsedSticks"
  [RawAngularRate] -> RawSensorsBus/2  "AngularRate"
  [JoystickPilot] -> CommandsBus/12  "Pilot"
  [RawAcceleration] -> RawSensorsBus/1  "Acceleration"
  [JoystickConnected] -> CommandsBus/5  "Connected"
  [PWMStatus] -> CommandsBus/3  "PWMStatus"
  [TimeSeconds] -> RawSensorsBus/4, HorizontalLogger50/1  "Time"
  TelemetryPacker50/3 -> RadioUSBTransport50/3  "SensorFrame246"
  [SchedulerStatus] -> ExtraSensorsBus/4  "Scheduler"
  [LogMagneticField] -> ExtraSensorsBus/2  "Mag"
  [HorizontalMotion] -> HorizontalLogger50/3
  [SamplePeriod] -> CommandsBus/9  "Dt"
  [LogFlowDistance50] -> HoldFlowDistance/1  "Distance50Hz"
  [HorizontalControlDiagnostics] -> HorizontalLogger50/2
  [FilteredAcceleration] -> EstimatesBus/6  "FilteredAccel"
  [ControlDiagnostics] -> EstimatesBus/4  "ControlDiagnostics"
  [AttitudeAngles] -> EstimatesBus/1  "Angles"
  [BottomDistanceMm] -> RawSensorsBus/5  "BottomMm"
  [CycleStartUs] -> CommandsBus/10  "StartUs"
  [AttitudeQuaternion] -> EstimatesBus/8  "Quaternion"
  [FilteredAngularRate] -> EstimatesBus/7  "FilteredGyro"
  [BottomRangeFresh] -> RawSensorsBus/6  "ToFFresh"
  [AppliedPWMCounts] -> CommandsBus/2  "AppliedCounts"
  [EstimatedAltitude] -> EstimatesBus/2  "Height"
  [BottomToFDiagnostics] -> RawSensorsBus/10  "ToFInfo"
  [BatteryVoltage] -> RawSensorsBus/8  "Voltage"
  [MotorDuty] -> CommandsBus/1  "Duty"
  [SensorFlags] -> EstimatesBus/9  "Flags"
  [IMUTemperature] -> RawSensorsBus/11  "Temperature"
  [PreviousMode] -> CommandsBus/7  "PreviousMode"
  [JoystickPacketError] -> CommandsBus/4  "PacketError"
  [VerticalVelocity] -> EstimatesBus/3  "Velocity"
  RadioUSBTransport50/2 -> RadioQueued/1  "RadioQueued"
  [AltitudeEnabled] -> CommandsBus/6  "AltitudeEnabled"
  RawSensorsBus/1 -> TelemetryPacker50/1  "RawSensors"
  MotorOutputEnabled/1 -> CommandsBus/13  "OutputEnabled"
  HorizontalLogger50/1 -> HorizontalFrameSent/1
  PreviousCycleTiming/1 -> ExtraSensorsBus/3  "Timing"
  HoldFlowDistance/1 -> ExtraSensorsBus/5  "Distance"
  EstimatesBus/1 -> TelemetryPacker50/2  "Estimates"
  CommandsBus/1 -> TelemetryPacker50/3  "Commands"
  ExtraSensorsBus/1 -> TelemetryPacker50/4  "ExtraSensors"
  TelemetryPacker50/1 -> RadioUSBTransport50/1  "SFI8Frame190"
  TelemetryPacker50/2 -> RadioUSBTransport50/2  "CommandFrame190"
  RadioUSBTransport50/1 -> USBDrops/1  "USBDrops"
  RadioUSBTransport50/3 -> LEDMode/1  "LEDMode"

== system Horizontal1804/EstimatorContext ==
  EstimatorFeedback : Inport
  BatteryVoltage : Inport  Port=2
  Dt : Inport  Port=3
  CorrectionContextInternal : BusCreator  Description=CorrectionContextInternal：異なる単位・型を持つ関連信号を名前付きバスにまとめます。入力線の信号名が項目名です。  Inputs=2
  EstimatorContextInternal : BusCreator  Description=EstimatorContextInternal：異なる単位・型を持つ関連信号を名前付きバスにまとめます。入力線の信号名が項目名です。  Inputs=6
  EstimatorFeedbackFields : BusSelector  Description=EstimatorFeedbackFields：バスから PreviousMode,AltitudeEnabled,AttitudeReset,ParkingReset を選びます。元のベクトルの成分順序は変更しません。  OutputSignals=PreviousMode,AltitudeEnabled,AttitudeReset,ParkingReset
  JapaneseExplanation : Subsystem  Description=前周期のモード、高度制御許可、姿勢・待機リセットを 1 周期保持して推定器へ渡します。状態更新順序と代数ループ回避に必要な遅延です。
      mask help: 前周期のモード、高度制御許可、姿勢・待機リセットを 1 周期保持して推定器へ渡します。状態更新順序と代数ループ回避に必要な遅延です。
      mask Display: disp(sprintf('前周期のモード、高度制御許可、姿勢・待機リセットを 1 周期保持して推定器へ渡します。\n状態更新順序と代数ループ回避に必要な遅延です。'));
  CorrectionContext : Outport
  EstimatorContext : Outport  Port=2
  wires:
  CorrectionContextInternal/1 -> CorrectionContext/1  "CorrectionContext"
  BatteryVoltage/1 -> EstimatorContextInternal/6
  EstimatorFeedbackFields/4 -> EstimatorContextInternal/5  "<ParkingReset>"
  Dt/1 -> CorrectionContextInternal/2, EstimatorContextInternal/3
  EstimatorFeedbackFields/2 -> EstimatorContextInternal/2  "<AltitudeEnabled>"
  EstimatorFeedback/1 -> EstimatorFeedbackFields/1
  EstimatorFeedbackFields/3 -> EstimatorContextInternal/4  "<AttitudeReset>"
  EstimatorFeedbackFields/1 -> EstimatorContextInternal/1, CorrectionContextInternal/1  "<PreviousMode>"
  EstimatorContextInternal/1 -> EstimatorContext/1  "EstimatorContext"

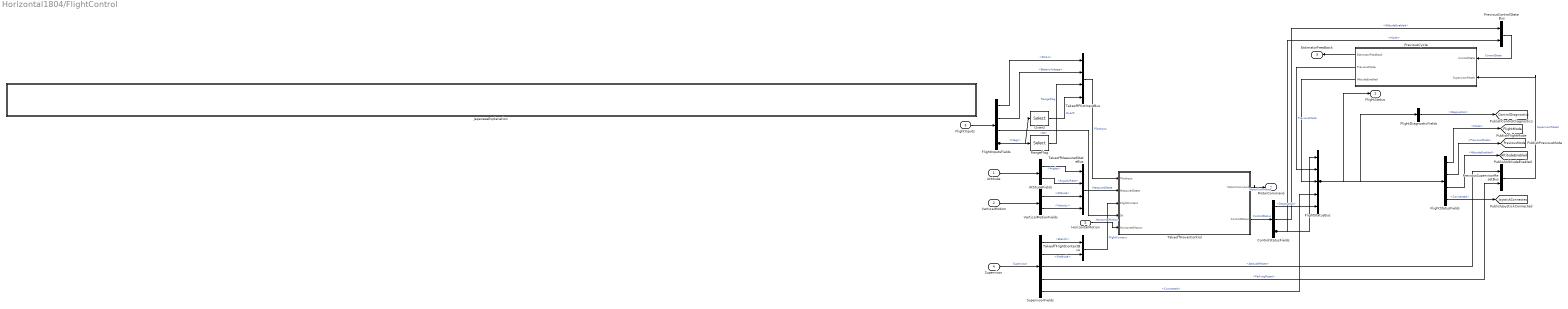
== system Horizontal1804/FlightControl ==
  Attitude : Inport
  VerticalMotion : Inport  Port=2
  FlightInputs : Inport  Port=3
  Supervisor : Inport  Port=4
  HorizontalMotion : Inport  Description=HorizontalMotion：水平推定・制御のデータと実行条件を選択・結合します。2軸の順序は局所X（基準機首）、Y（右）です。  Port=5  OutDataTypeStr=Bus: HorizontalMotionBus
  AttitudeFields : BusSelector  Description=AttitudeFields：バスから Angles,AngularRate を選びます。元のベクトルの成分順序は変更しません。  OutputSignals=Angles,AngularRate
  ControlStatusFields : BusSelector  Description=ControlStatusFields：バスから Diagnostics,AltitudeEnabled,Mode を選びます。元のベクトルの成分順序は変更しません。  OutputSignals=Diagnostics,AltitudeEnabled,Mode
  FlightDiagnosticFields : BusSelector  Description=FlightDiagnosticFields：バスから Diagnostics を選びます。元のベクトルの成分順序は変更しません。  OutputSignals=Diagnostics
  FlightInputsFields : BusSelector  Description=FlightInputsFields：バスから Sticks,BatteryVoltage,Dt,Flags を選びます。元のベクトルの成分順序は変更しません。  OutputSignals=Sticks,BatteryVoltage,Dt,Flags
  FlightStatusBus : BusCreator  Description=FlightStatusBus：異なる単位・型を持つ関連信号を名前付きバスにまとめます。入力線の信号名が項目名です。  Inputs=5
  FlightStatusFields : BusSelector  Description=FlightStatusFields：バスから Mode,PreviousMode,AltitudeEnabled,Connected を選びます。元のベクトルの成分順序は変更しません。  OutputSignals=Mode,PreviousMode,AltitudeEnabled,Connected
  JapaneseExplanation : Subsystem  Description=最上位 Stateflow の指令と姿勢・高度を受け、離着陸、7 個の PID、モーター配分を計算します。出力は Duty・PWM Counts、飛行状態、次周期の推定器コンテキストです。状態ログもこの階層に含みます。
      mask help: 最上位 Stateflow の指令と姿勢・高度を受け、離着陸、7 個の PID、モーター配分を計算します。出力は Duty・PWM Counts、飛行状態、次周期の推定器コンテキストです。状態ログもこの階層に含みます。
      mask Display: disp(sprintf('最上位 Stateflow の指令と姿勢・高度を受け、離着陸、7 個の PID、モーター配分を計算します。\n出力は Duty・PWM Counts、飛行状態、次周期の推定器コンテキストです。\n状態ログもこの階層に含みます。'));
  OverG : Selector  Description=OverG：必要なベクトル成分を選びます。選択位置は設定画面の Indices で確認します。  InputPortWidth=3  IndexOptions=Index vector (dialog)  Indices=1  OutputSizes=1
  PreviousControlStateBus : BusCreator  Description=PreviousControlStateBus：異なる単位・型を持つ関連信号を名前付きバスにまとめます。入力線の信号名が項目名です。  Inputs=2
  PreviousCycle : Subsystem  Description=前周期の推力・指令・モードなどを保持し、制御と次周期フィードバックへ渡します。Unit Delay は既存の更新順序を保つために必要です。
      mask help: 前周期の推力・指令・モードなどを保持し、制御と次周期フィードバックへ渡します。Unit Delay は既存の更新順序を保つために必要です。
      mask Display: disp('PreviousCycle');port_label('input',1,'ControlState');port_label('input',2,'SupervisorReset');port_label('output',1,'EstimatorFeedback');port_label('output',2,'PreviousMode');port_label('output',3,'AltitudeEnabled');
  PreviousSupervisorResetBus : BusCreator  Description=PreviousSupervisorResetBus：異なる単位・型を持つ関連信号を名前付きバスにまとめます。入力線の信号名が項目名です。  Inputs=2
  RangeFlag : Selector  Description=RangeFlag：必要なベクトル成分を選びます。選択位置は設定画面の Indices で確認します。  InputPortWidth=3  IndexOptions=Index vector (dialog)  Indices=2  OutputSizes=1
  SupervisorFields : BusSelector  Description=SupervisorFields：バスから Branch,PreMode,AttitudeReset,ParkingReset,Connected を選びます。元のベクトルの成分順序は変更しません。  OutputSignals=Branch,PreMode,AttitudeReset,ParkingReset,Connected
  TakeoffFlightContextBus : BusCreator  Description=TakeoffFlightContextBus：異なる単位・型を持つ関連信号を名前付きバスにまとめます。入力線の信号名が項目名です。  Inputs=2
  TakeoffHoverControl : Subsystem  Description=離着陸・高度制御・姿勢制御・角速度制御・モーター配分を機能別にまとめます。高度→速度、角度→角速度の二重ループを読みます。
      mask help: 離着陸・高度制御・姿勢制御・角速度制御・モーター配分を機能別にまとめます。高度→速度、角度→角速度の二重ループを読みます。
      mask Display: disp('TakeoffHoverControl');port_label('input',1,'PilotInput');port_label('input',2,'MeasuredState');port_label('input',3,'FlightContext');port_label('input',4,'Dt');port_label('input',5,'HorizontalMotion');port_label('output',1,'MotorCommand');port_label('output',2,'ControlStatus');
  TakeoffMeasuredStateBus : BusCreator  Description=TakeoffMeasuredStateBus：異なる単位・型を持つ関連信号を名前付きバスにまとめます。入力線の信号名が項目名です。  Inputs=4
  TakeoffPilotInputBus : BusCreator  Description=TakeoffPilotInputBus：異なる単位・型を持つ関連信号を名前付きバスにまとめます。入力線の信号名が項目名です。  Inputs=4
  VerticalMotionFields : BusSelector  Description=VerticalMotionFields：バスから Altitude,Velocity を選びます。元のベクトルの成分順序は変更しません。  OutputSignals=Altitude,Velocity
  MotorCommand : Outport
  FlightStatus : Outport  Port=2
  EstimatorFeedback : Outport  Port=3
  tag scope: AltitudeEnabled=global, ControlDiagnostics=global, FlightMode=global, JoystickConnected=global, PreviousMode=global
  wires:
  Supervisor/1 -> SupervisorFields/1  "Supervisor"
  VerticalMotion/1 -> VerticalMotionFields/1
  ControlStatusFields/2 -> PreviousControlStateBus/1  "<AltitudeEnabled>"
  Attitude/1 -> AttitudeFields/1
  FlightDiagnosticFields/1 -> [ControlDiagnostics]  "<Diagnostics>"
  FlightInputs/1 -> FlightInputsFields/1
  FlightInputsFields/3 -> TakeoffHoverControl/4(Dt)  "<Dt>"
  FlightStatusFields/4 -> [JoystickConnected]  "<Connected>"
  FlightInputsFields/1 -> TakeoffPilotInputBus/1  "<Sticks>"
  FlightInputsFields/4 -> RangeFlag/1, OverG/1  "<Flags>"
  FlightInputsFields/2 -> TakeoffPilotInputBus/2  "<BatteryVoltage>"
  OverG/1 -> TakeoffPilotInputBus/4  "OverG"
  VerticalMotionFields/2 -> TakeoffMeasuredStateBus/4  "<Velocity>"
  RangeFlag/1 -> TakeoffPilotInputBus/3  "RangeFlag"
  VerticalMotionFields/1 -> TakeoffMeasuredStateBus/3  "<Altitude>"
  AttitudeFields/1 -> TakeoffMeasuredStateBus/1  "<Angles>"
  AttitudeFields/2 -> TakeoffMeasuredStateBus/2  "<AngularRate>"
  TakeoffHoverControl/2(ControlStatus) -> ControlStatusFields/1  "ControlStatus"
  SupervisorFields/1 -> TakeoffFlightContextBus/1  "<Branch>"
  SupervisorFields/2 -> TakeoffFlightContextBus/2  "<PreMode>"
  PreviousSupervisorResetBus/1 -> PreviousCycle/2(SupervisorReset)  "SupervisorReset"
  SupervisorFields/3 -> PreviousSupervisorResetBus/1  "<AttitudeReset>"
  SupervisorFields/4 -> PreviousSupervisorResetBus/2  "<ParkingReset>"
  SupervisorFields/5 -> FlightStatusBus/4  "<Connected>"
  TakeoffPilotInputBus/1 -> TakeoffHoverControl/1(PilotInput)  "PilotInput"
  TakeoffFlightContextBus/1 -> TakeoffHoverControl/3(FlightContext)  "FlightContext"
  TakeoffMeasuredStateBus/1 -> TakeoffHoverControl/2(MeasuredState)  "MeasuredState"
  HorizontalMotion/1 -> TakeoffHoverControl/5(HorizontalMotion)  "HorizontalMotion"
  TakeoffHoverControl/1(MotorCommand) -> MotorCommand/1  "MotorCommand"
  ControlStatusFields/1 -> FlightStatusBus/5  "<Diagnostics>"
  ControlStatusFields/3 -> PreviousControlStateBus/2, FlightStatusBus/1  "<Mode>"
  FlightStatusBus/1 -> FlightDiagnosticFields/1, FlightStatus/1, FlightStatusFields/1
  FlightStatusFields/2 -> [PreviousMode]  "<PreviousMode>"
  PreviousCycle/3(AltitudeEnabled) -> FlightStatusBus/3
  FlightStatusFields/1 -> [FlightMode]  "<Mode>"
  PreviousCycle/2(PreviousMode) -> FlightStatusBus/2  "PreviousMode"
  PreviousCycle/1(EstimatorFeedback) -> EstimatorFeedback/1
  FlightStatusFields/3 -> [AltitudeEnabled]  "<AltitudeEnabled>"
  PreviousControlStateBus/1 -> PreviousCycle/1(ControlState)  "ControlState"

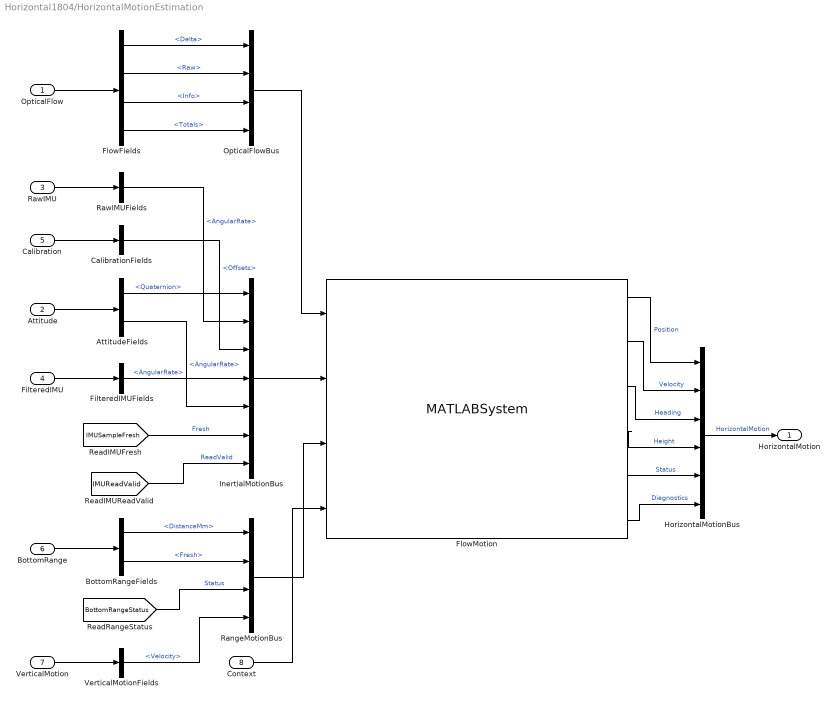
== system Horizontal1804/HorizontalMotionEstimation ==
  OpticalFlow : Inport  Description=OpticalFlow：水平推定・制御のデータと実行条件を選択・結合します。2軸の順序は局所X（基準機首）、Y（右）です。
  Attitude : Inport  Description=Attitude：水平推定・制御のデータと実行条件を選択・結合します。2軸の順序は局所X（基準機首）、Y（右）です。  Port=2
  RawIMU : Inport  Description=RawIMU：水平推定・制御のデータと実行条件を選択・結合します。2軸の順序は局所X（基準機首）、Y（右）です。  Port=3
  FilteredIMU : Inport  Description=FilteredIMU：水平推定・制御のデータと実行条件を選択・結合します。2軸の順序は局所X（基準機首）、Y（右）です。  Port=4
  Calibration : Inport  Description=Calibration：水平推定・制御のデータと実行条件を選択・結合します。2軸の順序は局所X（基準機首）、Y（右）です。  Port=5
  BottomRange : Inport  Description=BottomRange：水平推定・制御のデータと実行条件を選択・結合します。2軸の順序は局所X（基準機首）、Y（右）です。  Port=6
  VerticalMotion : Inport  Description=VerticalMotion：水平推定・制御のデータと実行条件を選択・結合します。2軸の順序は局所X（基準機首）、Y（右）です。  Port=7
  Context : Inport  Description=Context：水平推定・制御のデータと実行条件を選択・結合します。2軸の順序は局所X（基準機首）、Y（右）です。  Port=8
  AttitudeFields : BusSelector  Description=AttitudeFields：水平推定・制御のデータと実行条件を選択・結合します。2軸の順序は局所X（基準機首）、Y（右）です。  OutputSignals=Quaternion,AngularRate
  BottomRangeFields : BusSelector  Description=BottomRangeFields：水平推定・制御のデータと実行条件を選択・結合します。2軸の順序は局所X（基準機首）、Y（右）です。  OutputSignals=DistanceMm,Fresh
  CalibrationFields : BusSelector  Description=CalibrationFields：水平推定・制御のデータと実行条件を選択・結合します。2軸の順序は局所X（基準機首）、Y（右）です。  OutputSignals=Offsets
  FilteredIMUFields : BusSelector  Description=FilteredIMUFields：水平推定・制御のデータと実行条件を選択・結合します。2軸の順序は局所X（基準機首）、Y（右）です。  OutputSignals=AngularRate
  FlowFields : BusSelector  Description=FlowFields：水平推定・制御のデータと実行条件を選択・結合します。2軸の順序は局所X（基準機首）、Y（右）です。  OutputSignals=Delta,Raw,Info,Totals
  FlowMotion : MATLABSystem  Description=光学フロー・生角速度を同じ20 ms区間で集計し、ToF・姿勢・鉛直速度で床面へ投影します。投影高さ8 cm以上を観測し、品質・鮮度・傾き・速度の異常時は無効とします。局所Xは基準機首、Yは右です。  System=horizontal.FlowMotion  SampleTime=.0025  WindowSamples=8  XCountsPerRad=385  YCountsPerRad=385  MinQuality=25  MinHeightM=0.08  MaxHeightM=1.0  MaxRangeAgeS=.15  MaxFlowAgeS=.025  MaxSampleGapS=.01  MaxGyroAgeS=.0075  MaxSpeedMps=1.5  MaxVerticalSpeedMps=2.0  MaxTiltDeg=25  VelocityTimeConstantS=.05  SimulateUsing=Code generation
      mask Type: horizontal.FlowMotion
  HorizontalMotionBus : BusCreator  Description=HorizontalMotionBus：水平推定・制御のデータと実行条件を選択・結合します。2軸の順序は局所X（基準機首）、Y（右）です。  Inputs=6  OutDataTypeStr=Bus: HorizontalMotionBus  NonVirtualBus=on
      settings: InheritFromInputs=off
  InertialMotionBus : BusCreator  Description=InertialMotionBus：水平推定・制御のデータと実行条件を選択・結合します。2軸の順序は局所X（基準機首）、Y（右）です。  Inputs=7  OutDataTypeStr=Bus: HorizontalInertialBus  NonVirtualBus=on
      settings: InheritFromInputs=off
  OpticalFlowBus : BusCreator  Description=OpticalFlowBus：水平推定・制御のデータと実行条件を選択・結合します。2軸の順序は局所X（基準機首）、Y（右）です。  Inputs=4  OutDataTypeStr=Bus: HorizontalFlowBus  NonVirtualBus=on
      settings: InheritFromInputs=off
  RangeMotionBus : BusCreator  Description=RangeMotionBus：水平推定・制御のデータと実行条件を選択・結合します。2軸の順序は局所X（基準機首）、Y（右）です。  Inputs=4  OutDataTypeStr=Bus: HorizontalRangeBus  NonVirtualBus=on
      settings: InheritFromInputs=off
  RawIMUFields : BusSelector  Description=RawIMUFields：水平推定・制御のデータと実行条件を選択・結合します。2軸の順序は局所X（基準機首）、Y（右）です。  OutputSignals=AngularRate
  VerticalMotionFields : BusSelector  Description=VerticalMotionFields：水平推定・制御のデータと実行条件を選択・結合します。2軸の順序は局所X（基準機首）、Y（右）です。  OutputSignals=Velocity
  HorizontalMotion : Outport  Description=HorizontalMotion：水平推定・制御のデータと実行条件を選択・結合します。2軸の順序は局所X（基準機首）、Y（右）です。
  wires:
  FlowMotion/5 -> HorizontalMotionBus/5  "Status"
  VerticalMotion/1 -> VerticalMotionFields/1
  Calibration/1 -> CalibrationFields/1
  OpticalFlowBus/1 -> FlowMotion/1
  RawIMU/1 -> RawIMUFields/1
  FlowFields/2 -> OpticalFlowBus/2  "<Raw>"
  OpticalFlow/1 -> FlowFields/1
  FlowMotion/3 -> HorizontalMotionBus/3  "Heading"
  RangeMotionBus/1 -> FlowMotion/3
  BottomRange/1 -> BottomRangeFields/1
  FilteredIMU/1 -> FilteredIMUFields/1
  FlowFields/4 -> OpticalFlowBus/4  "<Totals>"
  Attitude/1 -> AttitudeFields/1
  FlowFields/1 -> OpticalFlowBus/1  "<Delta>"
  FlowFields/3 -> OpticalFlowBus/3  "<Info>"
  FlowMotion/6 -> HorizontalMotionBus/6  "Diagnostics"
  RawIMUFields/1 -> InertialMotionBus/2  "<AngularRate>"
  CalibrationFields/1 -> InertialMotionBus/3  "<Offsets>"
  [IMUReadValid] -> InertialMotionBus/7  "ReadValid"
  AttitudeFields/1 -> InertialMotionBus/1  "<Quaternion>"
  AttitudeFields/2 -> InertialMotionBus/5  "<AngularRate>"
  FilteredIMUFields/1 -> InertialMotionBus/4  "<AngularRate>"
  [IMUSampleFresh] -> InertialMotionBus/6  "Fresh"
  BottomRangeFields/1 -> RangeMotionBus/1  "<DistanceMm>"
  VerticalMotionFields/1 -> RangeMotionBus/4  "<Velocity>"
  BottomRangeFields/2 -> RangeMotionBus/2  "<Fresh>"
  HorizontalMotionBus/1 -> HorizontalMotion/1  "HorizontalMotion"
  [BottomRangeStatus] -> RangeMotionBus/3  "Status"
  InertialMotionBus/1 -> FlowMotion/2
  Context/1 -> FlowMotion/4
  FlowMotion/1 -> HorizontalMotionBus/1  "Position"
  FlowMotion/2 -> HorizontalMotionBus/2  "Velocity"
  FlowMotion/4 -> HorizontalMotionBus/4  "Height"

== system Horizontal1804/IMUSensor ==
  BMI270 : MATLABSystem  Description=BMI270の加速度・角速度・温度・Freshは従来と同じです。ReadValidは新規状態と独立したAPI読出し成功です。水平推定の短い再読出しと故障の判別に使います。  Priority=2  System=horizontal.IMUSource  SampleTime=0.0025  SimulateUsing=Code generation
      mask Type: horizontal.IMUSource
  JapaneseExplanation : Subsystem  Description=BMI270 の生加速度・角速度を XYZ のままバスへまとめます。センサー座標であり、単位は m/s²・rad/s。温度と Fresh は名前付き Goto でログへ公開します。
      mask help: BMI270 の生加速度・角速度を XYZ のままバスへまとめます。センサー座標であり、単位は m/s²・rad/s。温度と Fresh は名前付き Goto でログへ公開します。
      mask Display: disp(sprintf('BMI270 の生加速度・角速度を XYZ のままバスへまとめます。\nセンサー座標であり、単位は m/s²・rad/s。\n温度と Fresh は名前付き Goto でログへ公開します。'));
  RawIMUInternal : BusCreator  Description=RawIMUInternal：異なる単位・型を持つ関連信号を名前付きバスにまとめます。入力線の信号名が項目名です。  Inputs=2
  RawIMU : Outport
  tag scope: IMUReadValid=global, IMUSampleFresh=global, IMUTemperature=global, RawAcceleration=global, RawAngularRate=global
  wires:
  BMI270/5 -> [IMUReadValid]  "IMUReadValid"
  BMI270/4 -> [IMUSampleFresh]  "IMUFresh"
  BMI270/3 -> [IMUTemperature]  "Temperature"
  RawIMUInternal/1 -> RawIMU/1  "RawIMU"
  BMI270/2 -> [RawAngularRate], RawIMUInternal/2  "AngularRate"
  BMI270/1 -> [RawAcceleration], RawIMUInternal/1  "Acceleration"
